simulink model "test2"  (R2024b)
settings: Solver=VariableStepAuto  StartTime=0.0  StopTime=500  RelTol=1e-3
undefined symbols (not defined in the file or in its folder): RCAM_dynamics_fcn
settings Model: Creator=rukky  LastModifiedBy=kiriki

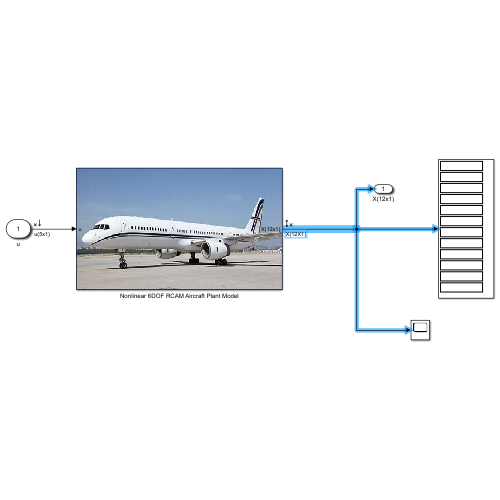
[thumbnail: Simulink's stored preview of the top-level diagram]
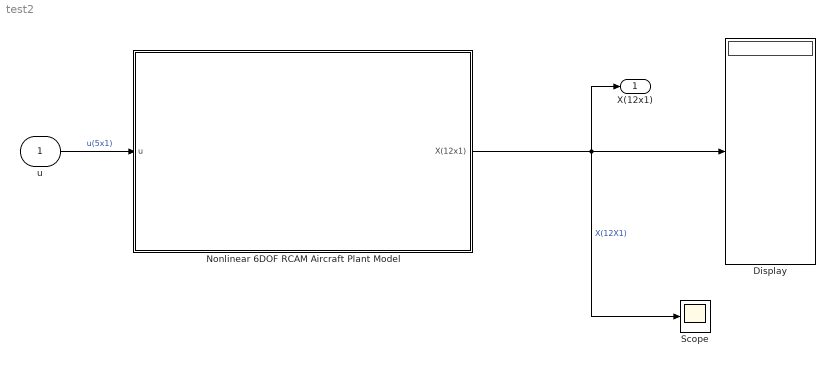
== system test2 ==
  u : Inport
  Display : Display
  Nonlinear 6DOF RCAM Aircraft Plant Model : Subsystem
      mask Display: image('$imagefile'); % Use "Edit Image" on toolstrip to change.
  Scope : Scope
  X(12x1) : Outport
  wires:
  Nonlinear 6DOF RCAM Aircraft Plant Model/1(X(12x1)) -> X(12x1)/1, Scope/1, Display/1  "X(12X1)"
  u/1 -> Nonlinear 6DOF RCAM Aircraft Plant Model/1(u)  "u(5x1)"

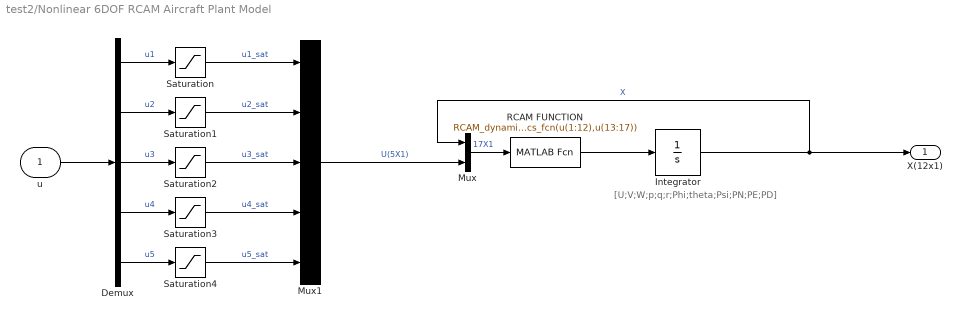
== system test2/Nonlinear 6DOF RCAM Aircraft Plant Model ==
  note: [U;V;W;p;q;r;Phi;theta;Psi;PN;PE;PD]
  u : Inport
  Demux : Demux  Outputs=5
  Integrator : Integrator  InitialCondition=|
      | [84.9905; 0;
      |  1.2713;
      | 0; 0; 0; 0; 0.1; 0; 0; 0.0149; 0]
  Mux : Mux  Inputs=2
  Mux1 : Mux  Inputs=5
  RCAM FUNCTION : MATLABFcn  MATLABFcn=RCAM_dynamics_fcn(u(1:12),u(13:17))
  Saturation : Saturate  UpperLimit=25*(pi/180)  LowerLimit=-15*(pi/180)
  Saturation1 : Saturate  UpperLimit=10*(pi/180)  LowerLimit=-25*(pi/180)
  Saturation2 : Saturate  UpperLimit=30*(pi/180)  LowerLimit=-30*(pi/180)
  Saturation3 : Saturate  UpperLimit=10*(pi/180)  LowerLimit=0.5*(pi/180)
  Saturation4 : Saturate  UpperLimit=10*(pi/180)  LowerLimit=0.5*(pi/180)
  X(12x1) : Outport
  wires:
  Integrator/1 -> Mux/1, X(12x1)/1  "X"
  u/1 -> Demux/1
  Demux/1 -> Saturation/1  "u1"
  Saturation/1 -> Mux1/1  "u1_sat"
  Demux/2 -> Saturation1/1  "u2"
  Demux/3 -> Saturation2/1  "u3"
  Demux/4 -> Saturation3/1  "u4"
  Demux/5 -> Saturation4/1  "u5"
  Saturation1/1 -> Mux1/2  "u2_sat"
  Saturation2/1 -> Mux1/3  "u3_sat"
  Saturation3/1 -> Mux1/4  "u4_sat"
  Saturation4/1 -> Mux1/5  "u5_sat"
  RCAM FUNCTION/1 -> Integrator/1
  Mux/1 -> RCAM FUNCTION/1  "17X1"
  Mux1/1 -> Mux/2  "U(5X1)"
